simulink model "SPIwork2"  (Simulink 7.3)
settings: Solver=FixedStepDiscrete  StartTime=0.0  StopTime=inf  FixedStep=.0002  RelTol=1e-3
undefined symbols (not defined in the file or in its folder): OC1max
libraries: dsPICdrivers x12
settings Model: Creator=ij8977  LastModifiedBy=ij8977  ExtModeTrigDuration=10000
settings SolverCC: PositivePriorityOrder=on
settings OptimizationCC: OptimizeModelRefInitCode=on  LifeSpan=1
settings HardwareCC: ProdBitPerInt=16  ProdEndianess=LittleEndian  ProdWordSize=16  ProdHWDeviceType=16-bit Generic
settings RTWCC: SystemTargetFile=dspic.tlc  TemplateMakefile=dspic_pic30_gcc.tmf  PostCodeGenCommand=dsPIC_Compile()  Description=Embedded Target for Microchip dsPIC (real-time)  ProcessScript=dspic_make_rtw_hook
settings CodeAppCC: IgnoreCustomStorageClasses=off
settings STFCustomTargetCC: ModelReferenceCompliant=off  IncludeMdlTerminateFcn=off  CombineOutputUpdateFcns=on  SuppressErrorStatus=on  ERTCustomFileBanners=on  SupportContinuousTime=off  SupportNonInlinedSFcns=off  SystemTargetFile=dspic.tlc
settings ERTTargetCC: MultiwordLength=2048  ModelReferenceCompliant=off  ParMdlRefBuildCompliant=off  CompOptLevelCompliant=off  IncludeMdlTerminateFcn=off  SuppressErrorStatus=on  ERTFirstTimeCompliant=off  ModelStepFunctionPrototypeControlCompliant=off  CPPClassGenCompliant=off  ExtModeMexFile=noextcomm  InlinedParameterPlacement=NonHierarchical  ERTSrcFileBannerTemplate=dsPIC_code_template.cgt  ERTHdrFileBannerTemplate=dsPIC_code_template.cgt  ERTDataSrcFileTemplate=dsPIC_code_template.cgt  ERTDataHdrFileTemplate=dsPIC_code_template.cgt  ERTCustomFileTemplate=dsPIC_main.tlc
settings CustomProperty: DataType=string  Value=C:\PROGRA~1\MATLAB\R2009a\bin\win32\gmake

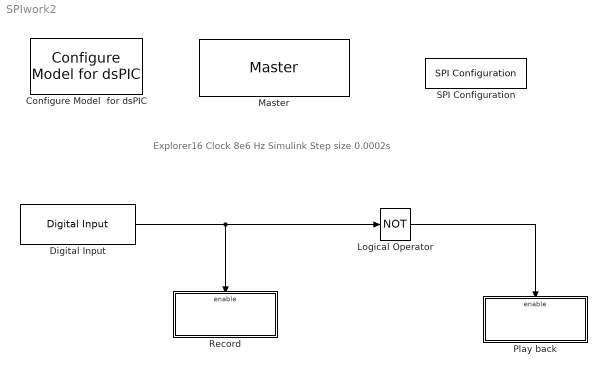
== system SPIwork2 ==
  note: Explorer16 Clock 8e6 Hz
      | Simulink Step size 0.0002s
  Configure Model  for dsPIC : dsPICdrivers/Simulink Configuration/Configure Model  for dsPIC
  Digital Input : dsPICdrivers/Digital I//O/Digital Input  Tag=dsPIC_Digital_Input  PORT=B  Pin=[1]  SampleTime=-1  OrderingInOutPopup=None
  Logical Operator : Logic  Operator=NOT  AllPortsSameDT=off  OutDataTypeMode=boolean  LogicDataType=fixdt(0, 8)  OutDataTypeStr=boolean
  Master : dsPICdrivers/Master  Tag=dsPIC_MASTER  Priority=1  TimeStepType=Timer1  picType=33fJ256MC710  fcy=40000000  Quartz_33f=8e6  PLLActive_33f=on  fcyDesired_33f=40000000  tmr1="[1  7999  0]"  tmr1Info="Time Step : 0.0002  ;   Error : 0%  PR1=7999"  tmr2345="[8  0  0  0  0  0  0  0]"  tmr2345cfg=[-1 -1 -1 -1 -1 -1 -1 -1]  IOautoConf=on  typePort="[ 0   0   0   0   0   0   0   0   0   0   0   0   0   0   0   0   0   0   0   0   0   0   0   0   0   0   0   0   0   0   0   0   0   0   0   0   0   0   0   0   0   0   0   0   0   0   0   0   0   0   0   0   0   0   0   0   0   6   0   0  21   0   0   0   0   0   0   0   0   0   0   0   0   0   0   0   0   0   0   0   0   0   0   0   0   0   0   0   0   0   0   0   0   0   0   0   0   0   0   0   0   0  17   0   0   0   0   0   0   0   0   0 ]"  TRIS="[ 65535  65535  65535  61439  65535  65535  65535 ]"  ADPCFG=0  MasterBusyPort=None  MasterOverloadPort=None  FOSC=Quartz (XT - HS)  ClockSwitchMonitor=Both disabled  TempProtection_33f=TEMP_ON  FPBOR=<empty>  PWRT=disable  MCLR=MCLR_DIS  PowerSave=off  OverrideFcy=off  NewFcy=1e6  PR2345="[65535  65535  65535  65535  65535  65535  65535  65535]"
  Play back : Subsystem  TreatAsAtomicUnit=on
  Record : Subsystem  TreatAsAtomicUnit=on
  SPI Configuration : dsPICdrivers/SPI PORT/SPI Configuration  Tag=dsPIC_config_SPI  Priority=2  ConfigurationTime=At boot time (only once)  OrderingInOutPopup=None  SampleTime=-1  Frame_Enable=0  Frame_Sync=None  SPI=2  MODE=MASTER  USER_SCALER=20  StartEnable=Enable  SDO_EN=off  DATA_LENGTH=8 bits  SS_EN=off  SMP=End of bit  CKP=high  CKE=Idle to Active  Status="OK - Mode 1  -    Fsck= 2000000Hz"
  wires:
  Digital Input/1 -> Logical Operator/1, Record/Enable
  Logical Operator/1 -> Play back/Enable

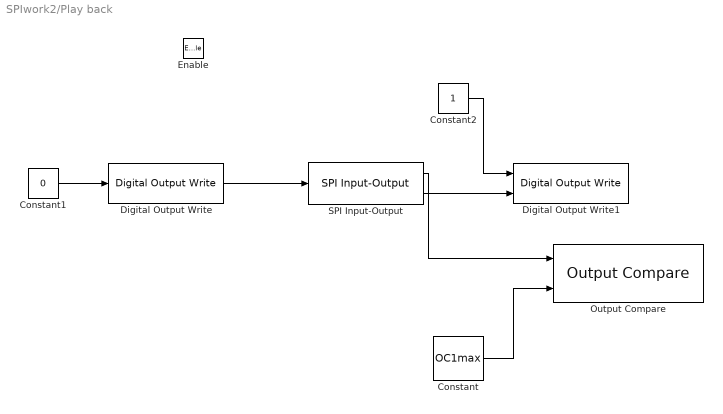
== system SPIwork2/Play back ==
  Enable : EnablePort
  Constant : Constant  Value=OC1max  OutDataTypeMode=uint16  OutDataType=fixdt(1, 16)  OutScaling=2^0  OutDataTypeStr=uint16
  Constant1 : Constant  Value=0  OutDataTypeMode=boolean  OutDataType=fixdt(1, 16)  OutScaling=2^0  OutDataTypeStr=boolean
  Constant2 : Constant  OutDataTypeMode=boolean  OutDataType=fixdt(1, 16)  OutScaling=2^0  OutDataTypeStr=boolean
  Digital Output Write : dsPICdrivers/Digital I//O/Digital Output Write  Tag=dsPIC_Digital_Output  Priority=5  PORT=D  Pin=[12]  Simultaneous=off  OrderingInOutPopup=Output
  Digital Output Write1 : dsPICdrivers/Digital I//O/Digital Output Write  Tag=dsPIC_Digital_Output  Priority=5  PORT=D  Pin=[12]  Simultaneous=off  OrderingInOutPopup=Input
  Output Compare : dsPICdrivers/Peripheral I//O/Output Compare  Tag=dsPIC_PWM_out  Priority=5  IntPriority=3  CHANNEL=[1]  Channel_UP_Down_Periode=[5]  MaxChannel=[0.02]  MaxName=' OC1max '  Precision=[9.9658]  Timer=[2]  Status=OK  SafeMarge=[0]  PortLetter=[68]  PortNumber=[0]  MaxValues=[9999]
  SPI Input-Output : dsPICdrivers/SPI PORT/SPI Input-Output  Tag=dsPIC_SPI  SPI=2  INPUT=on  RESET_INPUT=off  OUTPUT=off  SPECIAL_SPI=Re-Enable Execute and Disable  DATA_LENGTH=8 bits  WAIT_INPUTDATA=on  OrderingInOutPopup=Input & Output  SampleTime=-1
  wires:
  SPI Input-Output/1 -> Output Compare/1
  Constant/1 -> Output Compare/2
  Digital Output Write/1 -> SPI Input-Output/1
  Constant1/1 -> Digital Output Write/1
  Constant2/1 -> Digital Output Write1/1
  SPI Input-Output/2 -> Digital Output Write1/2

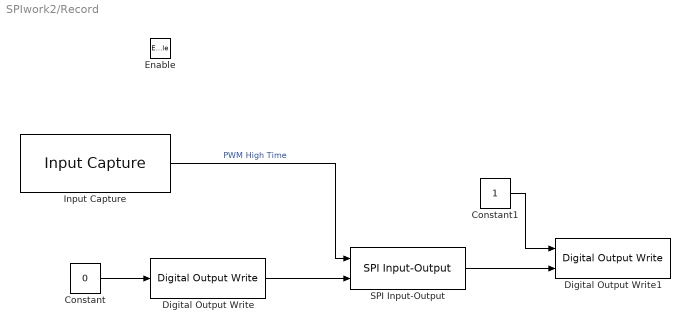
== system SPIwork2/Record ==
  Enable : EnablePort
  Constant : Constant  Value=0  OutDataTypeMode=boolean  OutDataType=fixdt(1, 16)  OutScaling=2^0  OutDataTypeStr=boolean
  Constant1 : Constant  OutDataTypeMode=boolean  OutDataType=fixdt(1, 16)  OutScaling=2^0  OutDataTypeStr=boolean
  Digital Output Write : dsPICdrivers/Digital I//O/Digital Output Write  Tag=dsPIC_Digital_Output  Priority=5  PORT=D  Pin=[12]  Simultaneous=off  OrderingInOutPopup=Output
  Digital Output Write1 : dsPICdrivers/Digital I//O/Digital Output Write  Tag=dsPIC_Digital_Output  Priority=5  PORT=D  Pin=[12]  Simultaneous=off  OrderingInOutPopup=Input
  Input Capture : dsPICdrivers/Peripheral I//O/Input Capture  Tag=dsPIC_PWM_IC  Priority=5  IntPriority=7  Channel=[ 2 ]  Channel_UP_Down_Periode=[1]  MaxChannel=[0.0025]  SafeMarge=[5]  MaxName=' IC2max '  Precision=[13.6798]  Timer=[2]  ChangeDetected=[0]  ChangeDetectedPortRef=3  SampleTime=-1  Status=OK
  SPI Input-Output : dsPICdrivers/SPI PORT/SPI Input-Output  Tag=dsPIC_SPI  SPI=2  INPUT=off  RESET_INPUT=off  OUTPUT=on  SPECIAL_SPI=Re-Enable Execute and Disable  DATA_LENGTH=8 bits  WAIT_INPUTDATA=on  OrderingInOutPopup=Input & Output  SampleTime=-1
  wires:
  Input Capture/1 -> SPI Input-Output/1  "PWM High Time"
  Digital Output Write/1 -> SPI Input-Output/2
  Constant/1 -> Digital Output Write/1
  SPI Input-Output/1 -> Digital Output Write1/2
  Constant1/1 -> Digital Output Write1/1
